simulink library "lib_AC_MGES"  (R2026a)
settings: Solver=VariableStepAuto
undefined symbols (not defined in the file): block_buses, block_fref, block_idx, block_toM, buses_lf, c_fd, c_kd1, c_kq1, c_kq2, fref, gen_static_params, Lbiginv, Lppd_pu, Lppq_pu, op_MGES, Ps_lf, Sb, T_meas_safe
(part 1 of 2)
settings Model: Creator=atomas  LastModifiedBy=atomas

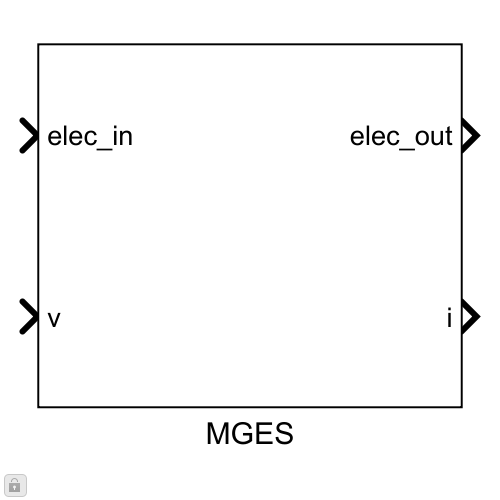
[thumbnail: Simulink's stored preview of the top-level diagram]
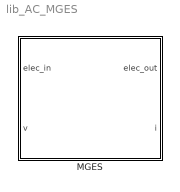
== system lib_AC_MGES ==
  MGES : Subsystem  mask(Synchronous machine){SGs_nodes=1, FBASE=50, D=0, H=3, Psimag_pu=0.8, Lssd_pu=0.1, Lssq_pu=0.1, Rs_pu=0.001, Lmd_pu=0.1, Lmq_pu=0.1, Rfd_pu=0.01, Lfd_pu=0.1, Rkd1_pu=1e6, Lkd1_pu=1e6, Rkd2_pu=1e6, Lkd2_pu=1e6, Rkq1_pu=1e6, Lkq1_pu=1e6, Rkq2_pu=1e6, Lkq2_pu=1e6, Rkq3_pu=1e6, Lkq3_pu=1e6, T_e=1, T_v=1, T_1=1, T_2=1, K_A=1, K_C=0, K_P=0, K_PR=1, K_IR=1, K_PM=1, K_IM=1, R_p=0.05, T_1g=1, T_2g=1, T_3=1, T_4=1, T_5=1, T_6=1, K_1=0, K_3=0, K_5=0, T_w1=1, T_w2=1, T_9=1, M=1, K_S1=0, T_1p=1, T_2p=1, T_3p=1, T_4p=1, T_7p=1, K_S2=1, K_S3=1, dynamic_stator=order 8, T_meas=0.01, cosn=1, T_w3=2}
      mask prompts: FBASE "Base frequency (Hz)"; D "Damping (pu)"; H "Inertia (s)"; Psimag_pu "Permanent flux (pu)"; Lssd_pu "Stator inductances (pu) Ld"; Lssq_pu "Stator inductances (pu) Lq"; Rs_pu "Stator resistances (pu)"; Lmd_pu "d-axis mutual inductance (pu)"; Lmq_pu "q-axis mutual inductance (pu)"; Rfd_pu "Excitation resistance (pu)"; Lfd_pu "Excitation inductance (pu)"; Rkd1_pu "d-axis damper resistance 1 (pu)"; Lkd1_pu "d-axis damper inductance 1 (pu)"; Rkd2_pu "d-axis damper resistance 2 (pu)"; Lkd2_pu "d-axis damper inductance 2 (pu)"; Rkq1_pu "q-axis damper resistance 1 (pu)"; Lkq1_pu "q-axis damper inductance 1 (pu)"; Rkq2_pu "q-axis damper resistance 2 (pu)"; Lkq2_pu "q-axis damper inductance 2 (pu)"; Rkq3_pu "q-axis damper resistance 3 (pu)"; Lkq3_pu "q-axis damper inductance 3 (pu)"; T_1p "T_1"; dynamic_stator "Electromagnetic complexity:"; T_meas "Governor speed measurement filter T_meas (s):"; cosn "Governor rated power factor cosn:"; T_w3 "PSS power washout time constant T_w3 (s):"
      mask help: Synchronous machine modelled in d-q reference frame.
      mask init:
      | [block_buses, block_idx, block_toM, block_fref, Lbiginv, Lssd_pu, Lssq_pu, Lmd_pu, Lmq_pu, Lfd_pu, Lkd1_pu, Lkd2_pu, Lkq1_pu, Lkq2_pu, Lkq3_pu, K_C, K_P, T_1, T_2, c_fd, c_kd1, Lppd_pu, c_kq1, c_kq2, Lppq_pu, stator_mode, use_Tmeas, use_PSS, use_LeadLag, use_KP, T_meas_safe, T_w3_safe, T_1_safe] = mask_init_MGES(gcb, Lssd_pu, Lssq_pu, Lmd_pu, Lmq_pu, Lfd_pu, Lkd1_pu, Lkd2_pu, Lkq1_pu, Lkq2_pu, Lkq3_pu, K_C, K_P, T_1, T_2, dynamic_stator, T_meas, K_S1, T_w3);
      mask Help: web([extractBefore(get_param(bdroot, 'filename'),gcs) 'Documentation/SM.html'])
      mask TypeOptions dynamic_stator: order 8 | order 4 | order 2
      mask DialogControl Params Prompt: Parameters
      mask DialogControl AVR Prompt: AVR
      mask DialogControl Gov Prompt: Speed governor
      mask DialogControl PSS Prompt: Power system stabiliser

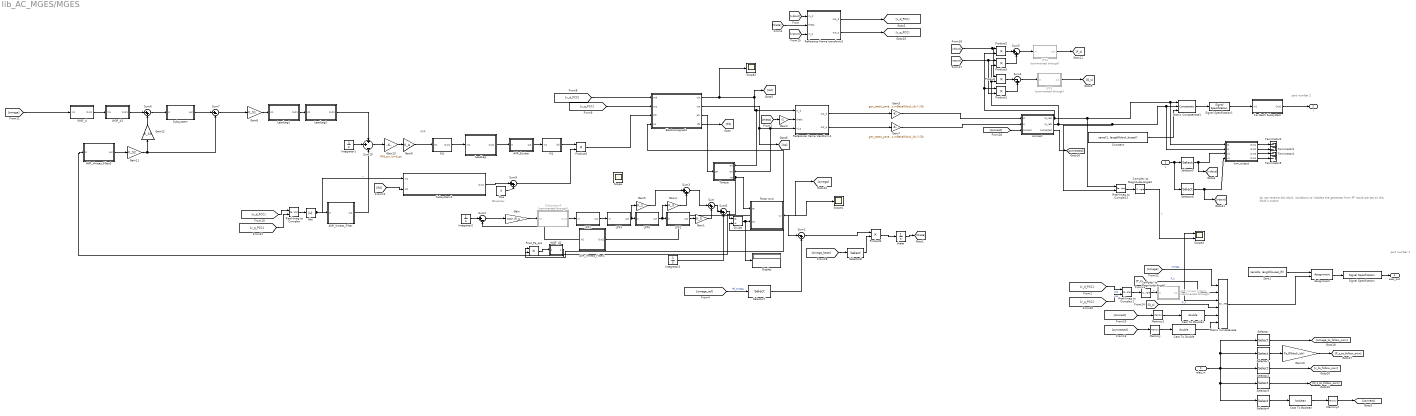
== system lib_AC_MGES/MGES ==
  note: Governor
  note: do not rename this block, conditions to initialise the generator from PF result are set on this block's output
  note: port number 1
  note: port number 2
  note: AVR
  elec_in : Inport
  v : Inport  Port=2
  AVR_Exciter : Subsystem  mask{T_s=T_e}
      mask prompts: T_s "Filter time constant"
  AVR_Vmeas_Filter : Subsystem  mask{T_r=T_v}
      mask prompts: T_r "Filter time constant"
  AVR_Vmeas_Filter1 : Subsystem  Variant=on
  AVR_Vmeas_Filter2 : Subsystem  Commented=through  mask{T_r=0.01}
      mask prompts: T_r "Filter time constant"
      mask Display:
      | try
      |     dpoly(1, [T_r, 1])
      | catch
      | end
  AVR_Vmeas_Filter3 : Subsystem  mask{T_r=T_7p}
      mask prompts: T_r "Filter time constant"
  Abs : Abs  SaturateOnIntegerOverflow=off
  Assignment : Assignment  NumberOfDimensions=2  DiagnosticForDimensions=Warning  IndexOptions=Assign all,Index vector (dialog)  Indices=1,block_idx  OutputSizes=1,1
  Cast To Boolean : DataTypeConversion  OutDataTypeStr=boolean  SaturateOnIntegerOverflow=off  RndMeth=Floor
  Cast To Double : DataTypeConversion  OutDataTypeStr=double  SaturateOnIntegerOverflow=off  RndMeth=Floor
  Cast To Double1 : DataTypeConversion  OutDataTypeStr=double  SaturateOnIntegerOverflow=off  RndMeth=Floor
  Complex to Magnitude-Angle1 : ComplexToMagnitudeAngle  Output=Magnitude
  Complex to Magnitude-Angle2 : ComplexToMagnitudeAngle  Output=Magnitude
  Constant : Constant  Value=zeros(1, length(block_buses))  VectorParams1D=off
  Display : Display
  Divide : Product  Inputs=*/
  Electromagnetic : Subsystem  Variant=on
  For Each Subsystem : Subsystem  TreatAsAtomicUnit=on
  Gain : Gain  Gain=cosn./R_p
  Gain1 : Gain  Gain=K_5
  Gain10 : Gain  Gain=Ps_lf(block_idx)
  Gain11 : Gain  Gain=K_S2
  Gain12 : Gain  Gain=K_S3
  Gain13 : Gain  Gain=Rfd_pu./Lmd_pu
  Gain2 : Gain  Gain=-1
  Gain3 : Gain  Gain=gen_static_params.mBase(block_idx)'./Sb
  Gain4 : Gain  Gain=K_3
  Gain5 : Gain  Gain=K_1
  Gain6 : Gain  Gain=K_A
  Gain7 : Gain  Gain=gen_static_params.mBase(block_idx)'./Sb
  Gain8 : Gain  Gain=K_S1
  Integrator1 : Integrator  InitialCondition=op_MGES.Integrator1
  Integrator2 : Integrator  InitialCondition=op_MGES.Integrator2
  Integrator3 : Integrator  InitialCondition=op_MGES.Integrator3
  LPF1 : Subsystem  mask{T_s=T_6}
      mask prompts: T_s "Filter time constant"
  LPF2 : Subsystem  mask{T_s=T_3}
      mask prompts: T_s "Filter time constant"
  LPF3 : Subsystem  mask{T_s=T_4}
      mask prompts: T_s "Filter time constant"
  LPF4 : Subsystem  Commented=through  mask{T_s=0.01}
      mask prompts: T_s "Filter time constant"
      mask Display:
      | try
      |     dpoly(1, [T_s, 1])
      | catch
      | end
  LPF5 : Subsystem  Commented=through  mask{T_s=0.01}
      mask prompts: T_s "Filter time constant"
      mask Display:
      | try
      |     dpoly(1, [T_s, 1])
      | catch
      | end
  LPF6 : Subsystem  mask{T_s=T_5}
      mask prompts: T_s "Filter time constant"
  LeadLag : Subsystem  Variant=on
  LeadLag1 : Subsystem  mask{T_2=T_1p, T_1=T_2p}
      mask help:
      | Transfer function:
      |
      |   1 + sT_2
      | ---------------
      |   1 + sT_1
  LeadLag2 : Subsystem  mask{T_2=T_3p, T_1=T_4p}
      mask help:
      | Transfer function:
      |
      |   1 + sT_2
      | ---------------
      |   1 + sT_1
  Matrix Concatenate : Concatenate  NumInputs=6  Mode=Multidimensional array
  Matrix Concatenate1 : Concatenate  NumInputs=3  Mode=Multidimensional array
  Memory : Memory  InitialCondition=1
  Memory1 : Memory  InitialCondition=1
  Memory2 : Memory  InitialCondition=1
  One : Constant  Value=0  OutDataTypeStr=Inherit: Inherit via back propagation
  PI1 : Subsystem
  PI2 : Subsystem
  Prod_Pe_pss : Product
  Product{,1..5} (6 alike) : Product
  Real-Imag to Complex : RealImagToComplex
  Real-Imag to Complex1 : RealImagToComplex
  Real-Imag to Complex2 : RealImagToComplex
  Reference frame transform1 : Subsystem
  Reference frame transform3 : Subsystem
  Rotor axis : Subsystem
  Scope : Scope
      settings: ActiveDisplayYMinimum=-1  ActiveDisplayYMaximum=1  DataLoggingVariableName=ScopeData13
  Scope1 : Scope
      settings: ActiveDisplayYMinimum=-0.058141408811601208  ActiveDisplayYMaximum=2.1702525958532117  DataLoggingVariableName=ScopeData3
  Scope2 : Scope
      settings: ActiveDisplayYMinimum=-0.402690614368146  ActiveDisplayYMaximum=1.3038964261892889  DataLoggingVariableName=ScopeData9
  Scope3 : Scope  NumInputPorts=2
      settings: ActiveDisplayYMinimum=0.29123  ActiveDisplayYMaximum=1.9416  DataLoggingVariableName=ScopeData3
  Selector : Selector  NumberOfDimensions=2  InputPortWidth=3  IndexOptions=Index vector (dialog),Index vector (dialog)  Indices=1,block_idx  OutputSizes=1,1
  Selector1 : Selector  NumberOfDimensions=2  InputPortWidth=3  IndexOptions=Index vector (dialog),Index vector (dialog)  Indices=2,block_idx  OutputSizes=1,1
  Selector2 : Selector  NumberOfDimensions=2  InputPortWidth=3  IndexOptions=Index vector (dialog),Index vector (dialog)  Indices=3,block_idx  OutputSizes=1,1
  Selector3 : Selector  NumberOfDimensions=2  InputPortWidth=3  IndexOptions=Index vector (dialog),Index vector (dialog)  Indices=4,block_idx  OutputSizes=1,1
  Selector4 : Selector  NumberOfDimensions=2  InputPortWidth=3  IndexOptions=Index vector (dialog),Index vector (dialog)  Indices=5,block_idx  OutputSizes=1,1
  Selector5 : Selector  NumberOfDimensions=2  InputPortWidth=3  IndexOptions=Index vector (dialog),Index vector (dialog)  Indices=1,block_buses  OutputSizes=1,1
  Selector6 : Selector  NumberOfDimensions=2  InputPortWidth=3  IndexOptions=Index vector (dialog),Index vector (dialog)  Indices=2,block_buses  OutputSizes=1,1
  Selector7 : Selector  InputPortWidth=length(fref.ref_units)  IndexOptions=Index vector (dialog)  Indices=block_fref  OutputSizes=1
  Selector8 : Selector  InputPortWidth=length(fref.ref_units)  IndexOptions=Index vector (dialog)  Indices=block_fref  OutputSizes=1
  Signal Specification : SignalSpecification  Dimensions=[6 length(buses_lf)]
  Signal Specification1 : SignalSpecification  Dimensions=[3 length(block_buses)]
  Subsystem : Subsystem
  Subsystem1 : Subsystem  Variant=on
  Subsystem4 : Subsystem  Commented=through  mask{T_2=T_2, T_1=T_1}
      mask help:
      | Transfer function:
      |
      |   1 + sT_2
      | ---------------
      |   1 + sT_1
  Sum{,3,5..6,8..9} (6 alike) : Sum  Inputs=|++
  Sum1 : Sum  Inputs=|-+
  Sum10 : Sum  Inputs=+|+|-
  Sum2 : Sum  Inputs=|+-
  Sum4 : Sum  Inputs=|-+
  Sum7 : Sum  Inputs=|+-
  Terminator{2..5} (4 alike) : Terminator
  Torque : Subsystem
      settings: PortSchema="{\"entries\":[{\"content\":{\"sides\":[{\"content\":{\"connectorIds\":[\"In1\"]},\"type\":\"ConnectorPlacement.EquallySpacedRectSide\",\"uuid\":\"b7abd3bc-22dd-4669-aa40-98bc76884565\"},{\"content\":{\"connectorIds\":[\"In2\",\"In3\",\"Out1\"],\"side\":\"RIGHT\"},\"type\":\"ConnectorPlacement.EquallySpacedRectSide\",\"uuid\":\"e9abb552-b46d-48ed-aa1f-0e9dac604fea\"},{\"content\":{\"connectorIds\":[],\"side\":\"TOP\"},\"type\":\"ConnectorPlacement.EquallySpacedRectSide\",\"uuid\":\"4b14997d-8f32-4cfb-8a1b-18cffb093d28\"}]},\"type\":\"ConnectorPlacement.EquallySpacedConnector\",\"uuid\":\"d6624493-e930-4f0d-8cbe-17f96cb72edc\"}],\"packageUris\":[\"http://schema.mathworks.com/mf0/Connector/R2020b\"],\"version\":\"1.0\"}"
  WOF_d : Subsystem
  WOF_d1 : Subsystem
  WOF_d2 : Subsystem  Variant=on
  Zero1 : Constant  Value=zeros(6, length(buses_lf))  VectorParams1D=off  OutDataTypeStr=Inherit: Inherit via back propagation
  connect : Subsystem
  theta : Integrator  InitialCondition=op_MGES.theta  UpperSaturationLimit=2*pi  LowerSaturationLimit=0
  trim_output : Subsystem
  elec_out : Outport
  i : Outport  Port=2
  wires:
  Subsystem1/1(Out1) -> Sum9/1
  [ifd] -> Subsystem1/2(In2)
  AVR_Vmeas_Filter/1(out) -> Sum10/3
  LeadLag/1(Out1) -> AVR_Exciter/1(in)
  PI2/1(Out1) -> LeadLag/1(In1)
  WOF_d2/1(Out1) -> AVR_Vmeas_Filter3/1(in)
  AVR_Vmeas_Filter1/1(Out1) -> Sum2/2
  Rotor axis/1(wr) -> AVR_Vmeas_Filter1/1(In1), Electromagnetic/4(ws), [omega], Scope1/1, Sum1/1, Divide/2, Prod_Pe_pss/2
  LPF5/1(out) -> [Q_s]
  Reference frame transform1/2(out_q) -> Gain7/1
  Product/1 -> Sum4/1
  Product1/1 -> Sum4/2
  theta/1 -> [theta]
  Gain2/1 -> Reference frame transform1/2(theta)
  [theta] -> Reference frame transform3/2(theta)
  LPF6/1(out) -> Gain4/1, LPF1/1(in)
  [theta] -> Gain2/1
  LPF2/1(out) -> LPF3/1(in)
  Sum4/1 -> LPF5/1(in)
  Sum5/1 -> LPF4/1(in)
  Product3/1 -> Sum5/2
  [omega_ref] -> Selector7/1  "ref_omega"
  Product2/1 -> Sum5/1
  Reference frame transform1/1(out_d) -> Gain3/1
  Subsystem4/1(Out1) -> LPF2/1(in)
  LPF4/1(out) -> [P_s]
  [P_s] -> Matrix Concatenate/2  "P_s"
  [omega] -> Matrix Concatenate/1  "omega"
  Complex to Magnitude-Angle1/1 -> AVR_Vmeas_Filter2/1(in)  "v"
  [Q_s] -> Matrix Concatenate/4  "Q_s"
  Selector3/1 -> [Q_s_to_follow_own]
  Selector/1 -> [omega_to_follow_own]
  Selector1/1 -> Gain10/1
  Selector2/1 -> [v_to_follow_own]
  [connect] -> Memory1/1
  [connected] -> Memory/1
  Cast To Double1/1 -> Matrix Concatenate/5
  Cast To Double/1 -> Matrix Concatenate/6
  Real-Imag to Complex1/1 -> Complex to Magnitude-Angle1/1
  [vdout] -> Product/1, Product2/1
  [vqout] -> Product3/1, Product1/2
  [v_d_PCC] -> Real-Imag to Complex1/1  "vod"
  [v_q_PCC] -> Real-Imag to Complex1/2  "voq"
  connect/3(connected) -> [connected]
  [connect] -> connect/3(connect)
  connect/1(id_real) -> Real-Imag to Complex2/1, trim_output/1(id), Matrix Concatenate1/1, Product1/1, Product2/2
  Selector4/1 -> Cast To Boolean/1
  Cast To Boolean/1 -> Memory2/1
  Zero1/1 -> Assignment/1
  Signal Specification/1 -> elec_out/1
  elec_in/1 -> Selector4/1, Selector3/1, Selector2/1, Selector1/1, Selector/1
  Assignment/1 -> Signal Specification/1
  Matrix Concatenate/1 -> Assignment/2
  Matrix Concatenate1/1 -> Signal Specification1/1
  Signal Specification1/1 -> For Each Subsystem/1(In1)
  Constant/1 -> Matrix Concatenate1/3
  For Each Subsystem/1(Out1) -> i/1
  connect/2(iq_real) -> Product3/2, Product/2, Real-Imag to Complex2/2, trim_output/2(iq), Matrix Concatenate1/2
  trim_output/3(Out3) -> Terminator4/1
  trim_output/1(Out1) -> Terminator2/1
  trim_output/4(Out4) -> Terminator5/1
  trim_output/2(Out2) -> Terminator3/1
  v/1 -> Selector6/1, Selector5/1
  Selector5/1 -> [vdout], trim_output/3(vd)
  Selector6/1 -> [vqout], trim_output/4(vq)
  [vqout] -> Reference frame transform3/3(in_q)
  [vdout] -> Reference frame transform3/1(in_d)
  Reference frame transform3/1(out_d) -> [v_d_PCC]
  Reference frame transform3/2(out_q) -> [v_q_PCC]
  Memory/1 -> Cast To Double/1
  Gain10/1 -> [P_s_to_follow_own]
  Memory1/1 -> Cast To Double1/1
  Memory2/1 -> [connect]
  Selector7/1 -> Sum1/2
  Selector8/1 -> Product4/2
  [omega_base] -> Selector8/1
  Product4/1 -> theta/1
  Sum1/1 -> Product4/1
  Gain/1 -> Subsystem4/1(In1)
  Sum2/1 -> Gain/1
  Integrator1/1 -> Sum10/2
  Gain6/1 -> PI2/1(In1)
  [v_d_PCC] -> Real-Imag to Complex/1
  Abs/1 -> AVR_Vmeas_Filter/1(in), Subsystem1/1(In1)  "v"
  [v_q_PCC] -> Real-Imag to Complex/2
  Real-Imag to Complex/1 -> Abs/1
  AVR_Vmeas_Filter2/1(out) -> Matrix Concatenate/3, Scope3/1
  Real-Imag to Complex2/1 -> Complex to Magnitude-Angle2/1
  Complex to Magnitude-Angle2/1 -> Scope3/2  "v"
  Electromagnetic/2(isq) -> [isq], Torque/3(isq), Reference frame transform1/3(in_q)
  Electromagnetic/1(isd) -> Scope2/1, Reference frame transform1/1(in_d), Torque/2(isd), [isd]
  [v_d_PCC] -> Electromagnetic/1(vsd)
  [v_q_PCC] -> Electromagnetic/2(vsq)
  Electromagnetic/3(psi) -> Torque/1(psi)
  Electromagnetic/4(ifd) -> [ifd]
  AVR_Exciter/1(out) -> PI1/1(In1)
  PI1/1(vfd) -> Product5/1
  LPF3/1(out) -> Gain5/1, LPF6/1(in)
  LPF1/1(out) -> Gain1/1
  Gain1/1 -> Sum/2
  Sum3/1 -> Sum/1
  Gain4/1 -> Sum3/2
  Gain5/1 -> Sum3/1
  Gain3/1 -> connect/1(id)
  Gain7/1 -> connect/2(iq)
  WOF_d/1(Out1) -> WOF_d1/1(In1)
  Gain8/1 -> LeadLag1/1(In1)
  LeadLag1/1(Out1) -> LeadLag2/1(In1)
  [omega] -> WOF_d/1(In1)
  WOF_d1/1(Out1) -> Sum6/1
  Sum6/1 -> Subsystem/1(in)
  Subsystem/1(out) -> Sum7/1
  Sum7/1 -> Gain8/1
  Gain12/1 -> Sum6/2
  Gain11/1 -> Sum7/2, Gain12/1
  AVR_Vmeas_Filter3/1(out) -> Gain11/1
  Integrator2/1 -> Sum2/1
  Torque/1(te) -> Rotor axis/1(te), Prod_Pe_pss/1
  Sum10/1 -> Gain13/1
  Gain13/1 -> Gain6/1
  Sum/1 -> Sum8/1
  Sum8/1 -> Divide/1
  Integrator3/1 -> Sum8/2
  LeadLag2/1(Out1) -> Sum10/1
  Divide/1 -> Display/1, Rotor axis/2(tm)
  Product5/1 -> Electromagnetic/3(vfd)
  Sum9/1 -> Product5/2
  One/1 -> Sum9/2
  Prod_Pe_pss/1 -> WOF_d2/1(In1)

== system lib_AC_MGES/MGES/AVR_Exciter ==
  in : Inport
  Gain : Gain  Gain=1./T_s
  Sum4 : Sum  Inputs=|+-
  x_a : Integrator  InitialCondition=op_MGES.AVR_Exciter_x_a
  out : Outport
  wires:
  Gain/1 -> x_a/1
  Sum4/1 -> Gain/1
  in/1 -> Sum4/1
  x_a/1 -> out/1, Sum4/2

== system lib_AC_MGES/MGES/AVR_Vmeas_Filter ==
  in : Inport
  Gain : Gain  Gain=1./T_r
  Sum4 : Sum  Inputs=|+-
  x_a : Integrator  InitialCondition=op_MGES.AVR_Vmeas_Filter_x_a
  out : Outport
  wires:
  Gain/1 -> x_a/1
  Sum4/1 -> Gain/1
  in/1 -> Sum4/1
  x_a/1 -> out/1, Sum4/2

== system lib_AC_MGES/MGES/AVR_Vmeas_Filter1 ==
  note: 1) Add Subsystem or Model blocks as valid variant choices.
      | 2) You cannot connect blocks at this level. At simulation, connectivity is automatically
      | determined, based on the active variant and port name matching.
  In1 : Inport
  Active : Subsystem  VariantControl=use_Tmeas == 1
  Bypass : Subsystem  VariantControl=(default)
  Out1 : Outport

== system lib_AC_MGES/MGES/AVR_Vmeas_Filter2 ==
  in : Inport
  Gain : Gain  Gain=1./T_r
  Sum4 : Sum  Inputs=|+-
  x_a : Integrator  InitialCondition=op_MGES.AVR_Vmeas_Filter2_x_a
  out : Outport
  wires:
  Gain/1 -> x_a/1
  Sum4/1 -> Gain/1
  in/1 -> Sum4/1
  x_a/1 -> out/1, Sum4/2

== system lib_AC_MGES/MGES/AVR_Vmeas_Filter3 ==
  in : Inport
  Gain : Gain  Gain=1./T_r
  Sum4 : Sum  Inputs=|+-
  x_a : Integrator  InitialCondition=op_MGES.AVR_Vmeas_Filter3_x_a
  out : Outport
  wires:
  x_a/1 -> Sum4/2, out/1
  in/1 -> Sum4/1
  Sum4/1 -> Gain/1
  Gain/1 -> x_a/1

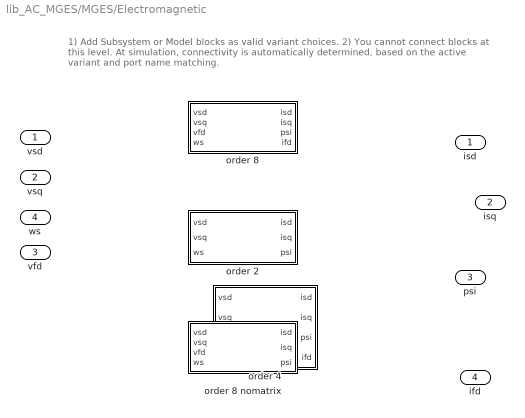
== system lib_AC_MGES/MGES/Electromagnetic ==
  note: 1) Add Subsystem or Model blocks as valid variant choices.
      | 2) You cannot connect blocks at this level. At simulation, connectivity is automatically
      | determined, based on the active variant and port name matching.
  vsd : Inport
  vsq : Inport  Port=2
  vfd : Inport  Port=3
  ws : Inport  Port=4
  order 2 : Subsystem  VariantControl=stator_mode == 2
  order 4 : Subsystem  VariantControl=stator_mode == 4
  order 8 : Subsystem  VariantControl=(default)
  order 8 nomatrix : Subsystem  VariantControl=stator_mode == 1  mask{Lssd_pu=Lssd_pu, Lssq_pu=Lssq_pu, Lmd_pu=Lmd_pu, Lmq_pu=Lmq_pu, Lfd_pu=Lfd_pu, Lkd1_pu=Lkd1_pu, Lkd2_pu=Lkd2_pu, Lkq1_pu=Lkq1_pu, Lkq2_pu=Lkq2_pu, Lkq3_pu=Lkq3_pu}
      mask init:
      | Matrix_flux_to_i = mask_init_order8_nomatrix(Lssd_pu, Lssq_pu, Lmd_pu, Lmq_pu, Lfd_pu, Lkd1_pu, Lkd2_pu, Lkq1_pu, Lkq2_pu, Lkq3_pu);
  isd : Outport
  isq : Outport  Port=2
  psi : Outport  Port=3
  ifd : Outport  Port=4

== system lib_AC_MGES/MGES/For Each Subsystem ==
  In1 : Inport  Partition=on  PartitionDimension=1  PartitionWidth=1  PartitionOffset=0
  For Each : ForEach  DisableCoverage=on
  State-Space : StateSpace  A=[]  B=[]  C=[]  D=block_toM  InitialCondition=0  ParameterTunability=Optimized
  Transpose : Math  Operator=transpose
  Transpose1 : Math  Operator=transpose
  Out1 : Outport  ConcatenationDimension=1
  wires:
  Transpose1/1 -> Out1/1
  In1/1 -> Transpose/1
  Transpose/1 -> State-Space/1
  State-Space/1 -> Transpose1/1

== system lib_AC_MGES/MGES/LPF1 ==
  in : Inport
  Gain : Gain  Gain=1./T_s
  Sum4 : Sum  Inputs=|+-
  x_a : Integrator  InitialConditionSource=external  InitialCondition=op_MGES.LPF1_x_a
  out : Outport
  wires:
  Gain/1 -> x_a/1
  Sum4/1 -> Gain/1
  in/1 -> x_a/2, Sum4/1
  x_a/1 -> out/1, Sum4/2

== system lib_AC_MGES/MGES/LPF2 ==
  in : Inport
  Gain : Gain  Gain=1./T_s
  Sum4 : Sum  Inputs=|+-
  x_a : Integrator  InitialConditionSource=external  InitialCondition=op_MGES.LPF2_x_a
  out : Outport
  wires:
  Gain/1 -> x_a/1
  Sum4/1 -> Gain/1
  in/1 -> x_a/2, Sum4/1
  x_a/1 -> out/1, Sum4/2

== system lib_AC_MGES/MGES/LPF3 ==
  in : Inport
  Gain : Gain  Gain=1./T_s
  Sum4 : Sum  Inputs=|+-
  x_a : Integrator  InitialConditionSource=external  InitialCondition=op_MGES.LPF3_x_a
  out : Outport
  wires:
  Gain/1 -> x_a/1
  Sum4/1 -> Gain/1
  in/1 -> x_a/2, Sum4/1
  x_a/1 -> out/1, Sum4/2

== system lib_AC_MGES/MGES/LPF4 ==
  in : Inport
  Gain : Gain  Gain=1./T_s
  Sum4 : Sum  Inputs=|+-
  x_a : Integrator  InitialCondition=op_MGES.LPF4_x_a
  out : Outport
  wires:
  x_a/1 -> Sum4/2, out/1
  in/1 -> Sum4/1
  Sum4/1 -> Gain/1
  Gain/1 -> x_a/1

== system lib_AC_MGES/MGES/LPF5 ==
  in : Inport
  Gain : Gain  Gain=1./T_s
  Sum4 : Sum  Inputs=|+-
  x_a : Integrator  InitialCondition=op_MGES.LPF5_x_a
  out : Outport
  wires:
  Gain/1 -> x_a/1
  Sum4/1 -> Gain/1
  in/1 -> Sum4/1
  x_a/1 -> out/1, Sum4/2

== system lib_AC_MGES/MGES/LPF6 ==
  in : Inport
  Gain : Gain  Gain=1./T_s
  Sum4 : Sum  Inputs=|+-
  x_a : Integrator  InitialConditionSource=external  InitialCondition=op_MGES.LPF6_x_a
  out : Outport
  wires:
  Gain/1 -> x_a/1
  Sum4/1 -> Gain/1
  in/1 -> x_a/2, Sum4/1
  x_a/1 -> out/1, Sum4/2

== system lib_AC_MGES/MGES/LeadLag ==
  note: 1) Add Subsystem or Model blocks as valid variant choices.
      | 2) You cannot connect blocks at this level. At simulation, connectivity is automatically
      | determined, based on the active variant and port name matching.
  In1 : Inport
  Active : Subsystem  VariantControl=use_LeadLag == 1
  Bypass : Subsystem  VariantControl=(default)
  Out1 : Outport

== system lib_AC_MGES/MGES/LeadLag1 ==
  In1 : Inport
  Gain : Gain  Gain=1./T_1
  Gain2 : Gain  Gain=T_2./T_1
  Sum : Sum  Inputs=|+-
  Sum1 : Sum  Inputs=++|
  x_f : Integrator  InitialConditionSource=external  InitialCondition=op_MGES.LeadLag1_x_f
  Out1 : Outport
  wires:
  x_f/1 -> Sum1/2, Sum/2
  Gain/1 -> x_f/1
  Sum/1 -> Gain/1, Gain2/1
  Gain2/1 -> Sum1/1
  Sum1/1 -> Out1/1
  In1/1 -> x_f/2, Sum/1

== system lib_AC_MGES/MGES/LeadLag2 ==
  In1 : Inport
  Gain : Gain  Gain=1./T_1
  Gain2 : Gain  Gain=T_2./T_1
  Sum : Sum  Inputs=|+-
  Sum1 : Sum  Inputs=++|
  x_f : Integrator  InitialConditionSource=external  InitialCondition=op_MGES.LeadLag2_x_f
  Out1 : Outport
  wires:
  In1/1 -> Sum/1, x_f/2
  Sum1/1 -> Out1/1
  Gain2/1 -> Sum1/1
  Sum/1 -> Gain2/1, Gain/1
  Gain/1 -> x_f/1
  x_f/1 -> Sum/2, Sum1/2

== system lib_AC_MGES/MGES/PI1 ==
  In1 : Inport
  Gain1 : Gain  Gain=K_IM ~= 0
  Gain4 : Gain  Gain=K_PM
  Gain5 : Gain  Gain=K_IM
  Integrator : Integrator  InitialCondition=op_MGES.PI1_Integrator
  Sum7 : Sum  Inputs=|++
  vfd : Outport
  wires:
  Integrator/1 -> Gain1/1
  Gain4/1 -> Sum7/1
  Sum7/1 -> vfd/1
  In1/1 -> Gain4/1, Gain5/1
  Gain5/1 -> Integrator/1
  Gain1/1 -> Sum7/2

== system lib_AC_MGES/MGES/PI2 ==
  In1 : Inport
  Gain1 : Gain  Gain=K_IR ~= 0
  Gain4 : Gain  Gain=K_PR
  Gain5 : Gain  Gain=K_IR
  Integrator : Integrator  InitialCondition=op_MGES.PI2_Integrator
  Sum7 : Sum  Inputs=|++
  Out1 : Outport
  wires:
  Integrator/1 -> Gain1/1
  Gain4/1 -> Sum7/1
  Sum7/1 -> Out1/1
  In1/1 -> Gain4/1, Gain5/1
  Gain5/1 -> Integrator/1
  Gain1/1 -> Sum7/2

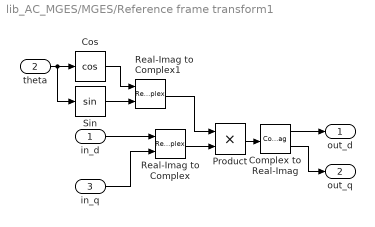
== system lib_AC_MGES/MGES/Reference frame transform1 ==
  in_d : Inport
  theta : Inport  Port=2
  in_q : Inport  Port=3
  Complex to Real-Imag : ComplexToRealImag
  Cos : Trigonometry  SCDEnableBlockLinearizationSpecification=on  Operator=cos
  Product : Product
  Real-Imag to Complex : RealImagToComplex
  Real-Imag to Complex1 : RealImagToComplex
  Sin : Trigonometry  SCDEnableBlockLinearizationSpecification=on
  out_d : Outport
  out_q : Outport  Port=2
  wires:
  in_d/1 -> Real-Imag to Complex/1
  in_q/1 -> Real-Imag to Complex/2
  Complex to Real-Imag/1 -> out_d/1
  Sin/1 -> Real-Imag to Complex1/2
  Cos/1 -> Real-Imag to Complex1/1
  theta/1 -> Cos/1, Sin/1
  Product/1 -> Complex to Real-Imag/1
  Real-Imag to Complex/1 -> Product/2
  Real-Imag to Complex1/1 -> Product/1
  Complex to Real-Imag/2 -> out_q/1

== system lib_AC_MGES/MGES/Reference frame transform3 ==
  in_d : Inport
  theta : Inport  Port=2
  in_q : Inport  Port=3
  Complex to Real-Imag : ComplexToRealImag
  Cos : Trigonometry  SCDEnableBlockLinearizationSpecification=on  Operator=cos
  Product : Product
  Real-Imag to Complex : RealImagToComplex
  Real-Imag to Complex1 : RealImagToComplex
  Sin : Trigonometry  SCDEnableBlockLinearizationSpecification=on
  out_d : Outport
  out_q : Outport  Port=2
  wires:
  Complex to Real-Imag/2 -> out_q/1
  Real-Imag to Complex1/1 -> Product/1
  Real-Imag to Complex/1 -> Product/2
  Product/1 -> Complex to Real-Imag/1
  theta/1 -> Sin/1, Cos/1
  Cos/1 -> Real-Imag to Complex1/1
  Sin/1 -> Real-Imag to Complex1/2
  Complex to Real-Imag/1 -> out_d/1
  in_q/1 -> Real-Imag to Complex/2
  in_d/1 -> Real-Imag to Complex/1

== system lib_AC_MGES/MGES/Rotor axis ==
  te : Inport
  tm : Inport  Port=2
  Gain : Gain  Gain=1./(2*H)
  Gain1 : Gain  Gain=D
  Sum1 : Sum  Inputs=+|-|-  InputSameDT=on  SaturateOnIntegerOverflow=on  OutDataTypeStr=Inherit: Same as first input
  \omega_r : Integrator  InitialCondition=op_MGES.Rotor_axis_omega_r  UpperSaturationLimit=2*pi  LowerSaturationLimit=0
  wr : Outport  VectorParamsAs1DForOutWhenUnconnected=off
  wires:
  tm/1 -> Sum1/1
  \omega_r/1 -> wr/1, Gain1/1
  te/1 -> Sum1/2
  Sum1/1 -> Gain/1
  Gain/1 -> \omega_r/1
  Gain1/1 -> Sum1/3

== system lib_AC_MGES/MGES/Subsystem ==
  in : Inport
  LPF1 : Subsystem  mask{T_s=T_9}
      mask prompts: T_s "Filter time constant"
  LPF2 : Subsystem  mask{T_s=T_9}
      mask prompts: T_s "Filter time constant"
  LPF3 : Subsystem  mask{T_s=T_9}
      mask prompts: T_s "Filter time constant"
  LPF4 : Subsystem  mask{T_s=T_9}
      mask prompts: T_s "Filter time constant"
  LPF7 : Subsystem  mask{T_s=T_9}
      mask prompts: T_s "Filter time constant"
  out : Outport
  wires:
  LPF2/1(out) -> LPF3/1(in)
  LPF3/1(out) -> LPF4/1(in)
  LPF7/1(out) -> LPF1/1(in)
  LPF4/1(out) -> out/1
  LPF1/1(out) -> LPF2/1(in)
  in/1 -> LPF7/1(in)

== system lib_AC_MGES/MGES/Subsystem1 ==
  note: 1) Add Subsystem or Model blocks as valid variant choices.
      | 2) You cannot connect blocks at this level. At simulation, connectivity is automatically
      | determined, based on the active variant and port name matching.
  In1 : Inport
  In2 : Inport  Port=2
  Active : Subsystem  VariantControl=use_KP == 1
  Bypass : Subsystem  VariantControl=(default)
  Out1 : Outport

== system lib_AC_MGES/MGES/Subsystem4 ==
  In1 : Inport
  Gain : Gain  Gain=1./T_1
  Gain2 : Gain  Gain=T_2./T_1
  Sum : Sum  Inputs=|+-
  Sum1 : Sum  Inputs=++|
  x_f : Integrator  InitialCondition=op_MGES.Subsystem4_x_f
  Out1 : Outport
  wires:
  x_f/1 -> Sum1/2, Sum/2
  Gain/1 -> x_f/1
  Sum/1 -> Gain/1, Gain2/1
  Gain2/1 -> Sum1/1
  Sum1/1 -> Out1/1
  In1/1 -> Sum/1

== system lib_AC_MGES/MGES/Torque ==
  psi : Inport
  isd : Inport  Port=2
  isq : Inport  Port=3
  Product1 : Product
  Product2 : Product
  Selector : Selector  NumberOfDimensions=2  InputPortWidth=9  IndexOptions=Index vector (dialog),Select all  Indices=[1],1  OutputSizes=1,1
  Selector1 : Selector  NumberOfDimensions=2  InputPortWidth=9  IndexOptions=Index vector (dialog),Select all  Indices=[2],1  OutputSizes=1,1
  Sum : Sum  Inputs=+||-
  te : Outport  VectorParamsAs1DForOutWhenUnconnected=off
  wires:
  Product1/1 -> Sum/1
  Sum/1 -> te/1
  Selector/1 -> Product1/1  "psistatordq"
  psi/1 -> Selector1/1, Selector/1
  Product2/1 -> Sum/2
  isq/1 -> Product1/2
  isd/1 -> Product2/1
  Selector1/1 -> Product2/2  "psistatordq"

== system lib_AC_MGES/MGES/WOF_d ==
  In1 : Inport
  Gain : Gain  Gain=1./T_w1
  I : Integrator  InitialConditionSource=external  InitialCondition=op_MGES.WOF_d_I
  Sum : Sum  Inputs=+-|
  Sum4 : Sum  Inputs=|+-
  Out1 : Outport
  wires:
  Sum/1 -> Out1/1
  I/1 -> Sum/2, Sum4/2
  In1/1 -> Sum4/1, Sum/1, I/2
  Sum4/1 -> Gain/1
  Gain/1 -> I/1

== system lib_AC_MGES/MGES/WOF_d1 ==
  In1 : Inport
  Gain : Gain  Gain=1./T_w2
  I : Integrator  InitialConditionSource=external  InitialCondition=op_MGES.WOF_d1_I
  Sum : Sum  Inputs=+-|
  Sum4 : Sum  Inputs=|+-
  Out1 : Outport
  wires:
  Sum/1 -> Out1/1
  I/1 -> Sum/2, Sum4/2
  In1/1 -> Sum4/1, Sum/1, I/2
  Sum4/1 -> Gain/1
  Gain/1 -> I/1

== system lib_AC_MGES/MGES/WOF_d2 ==
  note: 1) Add Subsystem or Model blocks as valid variant choices.
      | 2) You cannot connect blocks at this level. At simulation, connectivity is automatically
      | determined, based on the active variant and port name matching.
  In1 : Inport
  Active : Subsystem  VariantControl=use_PSS == 1
  Bypass : Subsystem  VariantControl=(default)
  Out1 : Outport

== system lib_AC_MGES/MGES/connect ==
  id : Inport
  iq : Inport  Port=2
  connect : Inport  Port=3
  Switch : Switch  Criteria=u2 > Threshold  ZeroCross=off  SaturateOnIntegerOverflow=off  InputSameDT=off
  Switch1 : Switch  Criteria=u2 > Threshold  ZeroCross=off  SaturateOnIntegerOverflow=off  InputSameDT=off
  Zero1 : Constant  Value=0  VectorParams1D=off  OutDataTypeStr=Inherit: Inherit via back propagation
  Zero2 : Constant  Value=0  VectorParams1D=off  OutDataTypeStr=Inherit: Inherit via back propagation
  id_real : Outport
  iq_real : Outport  Port=2
  connected : Outport  Port=3  OutDataTypeStr=boolean
  wires:
  Switch/1 -> id_real/1
  Zero1/1 -> Switch/3
  id/1 -> Switch/1
  connect/1 -> connected/1, Switch1/2, Switch/2
  Switch1/1 -> iq_real/1
  iq/1 -> Switch1/1
  Zero2/1 -> Switch1/3

== system lib_AC_MGES/MGES/trim_output ==
  id : Inport
  iq : Inport  Port=2
  vd : Inport  Port=3
  vq : Inport  Port=4
  Out1 : Outport
  Out2 : Outport  Port=2
  Out3 : Outport  Port=3
  Out4 : Outport  Port=4
  wires:
  id/1 -> Out1/1
  vq/1 -> Out4/1
  vd/1 -> Out3/1
  iq/1 -> Out2/1

== system lib_AC_MGES/MGES/AVR_Vmeas_Filter1/Active ==
  In1 : Inport
  Impl : Subsystem  mask{T_r=T_meas_safe}
      mask prompts: T_r "Filter time constant"
  Out1 : Outport
  wires:
  Impl/1(out) -> Out1/1
  In1/1 -> Impl/1(in)

== system lib_AC_MGES/MGES/AVR_Vmeas_Filter1/Bypass ==
  In1 : Inport
  Out1 : Outport
  wires:
  In1/1 -> Out1/1

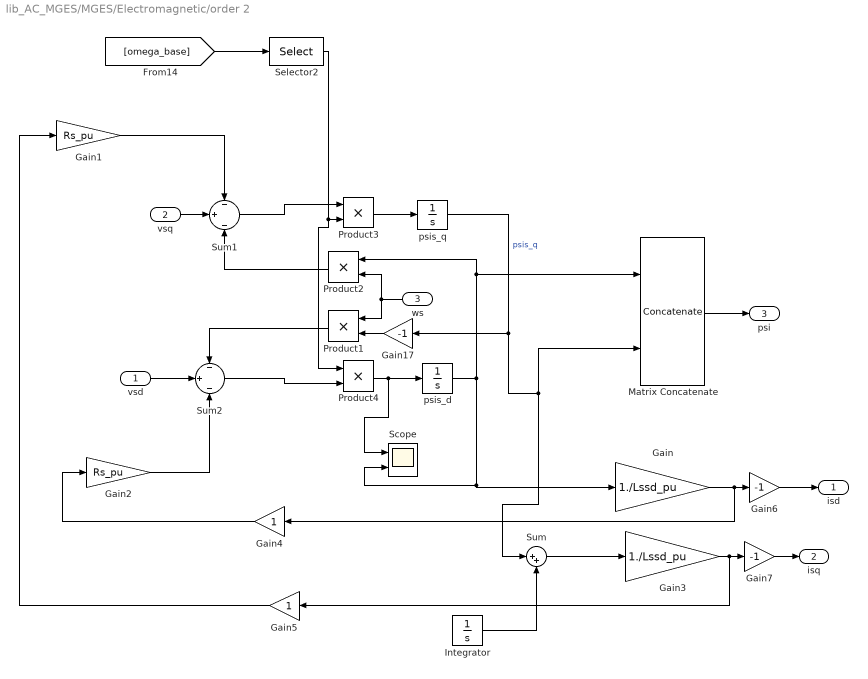
== system lib_AC_MGES/MGES/Electromagnetic/order 2 ==
  vsd : Inport
  vsq : Inport  Port=2
  ws : Inport  Port=3
  Gain : Gain  Gain=1./Lssd_pu
  Gain1 : Gain  Gain=Rs_pu
  Gain17 : Gain  Gain=-1
  Gain2 : Gain  Gain=Rs_pu
  Gain3 : Gain  Gain=1./Lssd_pu
  Gain4 : Gain
  Gain5 : Gain
  Gain6 : Gain  Gain=-1
  Gain7 : Gain  Gain=-1
  Integrator : Integrator  InitialCondition=op_MGES.Electromagnetic_order_2_Integrator
  Matrix Concatenate : Concatenate  Mode=Multidimensional array
  Product{1..4} (4 alike) : Product
  Scope : Scope  NumInputPorts=2
      settings: ActiveDisplayYMinimum=-176.647  ActiveDisplayYMaximum=19.6557
  Selector2 : Selector  InputPortWidth=length(fref.ref_units)  IndexOptions=Index vector (dialog)  Indices=block_fref  OutputSizes=1
  Sum : Sum  Inputs=|++
  Sum1 : Sum  Inputs=-|+|-  InputSameDT=on  SaturateOnIntegerOverflow=on  OutDataTypeStr=Inherit: Same as first input
  Sum2 : Sum  Inputs=-|+|-  InputSameDT=on  SaturateOnIntegerOverflow=on  OutDataTypeStr=Inherit: Same as first input
  psis_d : Integrator  InitialCondition=op_MGES.Electromagnetic_order_2_psis_d
  psis_q : Integrator  InitialCondition=op_MGES.Electromagnetic_order_2_psis_q
  isd : Outport  VectorParamsAs1DForOutWhenUnconnected=off
  isq : Outport  Port=2  VectorParamsAs1DForOutWhenUnconnected=off
  psi : Outport  Port=3  VectorParamsAs1DForOutWhenUnconnected=off
  wires:
  Product4/1 -> Scope/1, psis_d/1
  vsd/1 -> Sum2/2
  ws/1 -> Product1/1, Product2/2
  Matrix Concatenate/1 -> psi/1
  Product3/1 -> psis_q/1
  Sum1/1 -> Product3/1
  Product1/1 -> Sum2/1
  Product2/1 -> Sum1/3
  Sum2/1 -> Product4/2
  psis_q/1 -> Sum/1, Matrix Concatenate/2, Gain17/1  "psis_q"
  Gain1/1 -> Sum1/1
  [omega_base] -> Selector2/1
  vsq/1 -> Sum1/2
  Gain/1 -> Gain4/1, Gain6/1
  Gain2/1 -> Sum2/3
  Gain3/1 -> Gain5/1, Gain7/1
  Gain17/1 -> Product1/2
  Selector2/1 -> Product4/1, Product3/2
  Sum/1 -> Gain3/1
  Integrator/1 -> Sum/2
  Gain4/1 -> Gain2/1
  Gain5/1 -> Gain1/1
  psis_d/1 -> Product2/1, Matrix Concatenate/1, Gain/1, Scope/2
  Gain6/1 -> isd/1
  Gain7/1 -> isq/1

== system lib_AC_MGES/MGES/Electromagnetic/order 4 ==
  vsd : Inport
  vsq : Inport  Port=2
  vfd : Inport  Port=3
  ws : Inport  Port=4
  Stator circuit : Subsystem
  psi->i : Subsystem
  isd : Outport
  isq : Outport  Port=2
  psi : Outport  Port=3
  ifd : Outport  Port=4
  wires:
  psi->i/4(ifd) -> ifd/1
  psi->i/1(isd) -> isd/1
  vfd/1 -> Stator circuit/5(vfd)
  Stator circuit/1(psi) -> psi->i/1(psi), psi/1
  ws/1 -> Stator circuit/4(ws)
  vsq/1 -> Stator circuit/2(vsq)
  vsd/1 -> Stator circuit/1(vsd)
  psi->i/2(i) -> Stator circuit/3(i)
  psi->i/3(isq) -> isq/1

== system lib_AC_MGES/MGES/Electromagnetic/order 8 ==
  vsd : Inport
  vsq : Inport  Port=2
  vfd : Inport  Port=3
  ws : Inport  Port=4
  Stator circuit : Subsystem
  psi->i : Subsystem
  isd : Outport
  isq : Outport  Port=2
  psi : Outport  Port=3
  ifd : Outport  Port=4
  wires:
  psi->i/3(isq) -> isq/1
  psi->i/2(i) -> Stator circuit/3(i)
  vsd/1 -> Stator circuit/1(vsd)
  vsq/1 -> Stator circuit/2(vsq)
  ws/1 -> Stator circuit/4(ws)
  Stator circuit/1(psi) -> psi/1, psi->i/1(psi)
  vfd/1 -> Stator circuit/5(vfd)
  psi->i/1(isd) -> isd/1
  psi->i/4(ifd) -> ifd/1

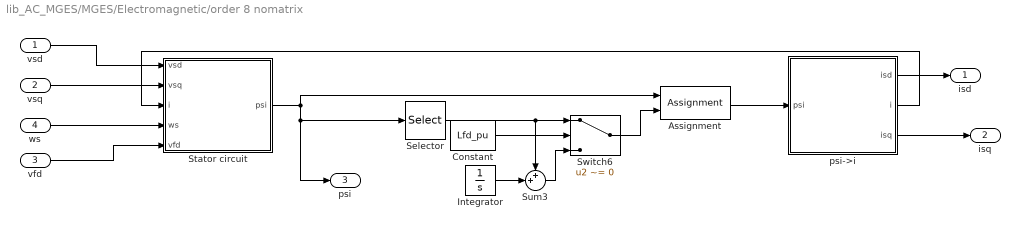
== system lib_AC_MGES/MGES/Electromagnetic/order 8 nomatrix ==
  vsd : Inport
  vsq : Inport  Port=2
  vfd : Inport  Port=3
  ws : Inport  Port=4
  Assignment : Assignment  NumberOfDimensions=2  DiagnosticForDimensions=Warning  IndexOptions=Index vector (dialog),Assign all  Indices=2,1  OutputSizes=1,1
  Constant : Constant  Value=Lfd_pu  VectorParams1D=off
  Integrator : Integrator  InitialCondition=op_MGES.Electromagnetic_order_8_nomatrix_Integrator
  Selector : Selector  NumberOfDimensions=2  InputPortWidth=3  IndexOptions=Index vector (dialog),Select all  Indices=2,1  OutputSizes=1,1
  Stator circuit : Subsystem
  Sum3 : Sum  Inputs=++|
  Switch6 : Switch  Criteria=u2 ~= 0  SaturateOnIntegerOverflow=off  InputSameDT=off
  psi->i : Subsystem
  isd : Outport
  isq : Outport  Port=2
  psi : Outport  Port=3
  wires:
  psi->i/3(isq) -> isq/1
  psi->i/2(i) -> Stator circuit/3(i)
  vsd/1 -> Stator circuit/1(vsd)
  vsq/1 -> Stator circuit/2(vsq)
  ws/1 -> Stator circuit/4(ws)
  Stator circuit/1(psi) -> psi/1, Selector/1, Assignment/1
  vfd/1 -> Stator circuit/5(vfd)
  psi->i/1(isd) -> isd/1
  Sum3/1 -> Switch6/3
  Constant/1 -> Switch6/2
  Integrator/1 -> Sum3/2
  Assignment/1 -> psi->i/1(psi)
  Selector/1 -> Sum3/1, Switch6/1
  Switch6/1 -> Assignment/2

== system lib_AC_MGES/MGES/LeadLag/Active ==
  In1 : Inport
  Impl : Subsystem
  Out1 : Outport
  wires:
  Impl/1(Out1) -> Out1/1
  In1/1 -> Impl/1(In1)

== system lib_AC_MGES/MGES/LeadLag/Bypass ==
  In1 : Inport
  Out1 : Outport
  wires:
  In1/1 -> Out1/1

== system lib_AC_MGES/MGES/Subsystem/LPF1 ==
  in : Inport
  Gain : Gain  Gain=1./T_s
  Sum4 : Sum  Inputs=|+-
  x_a : Integrator  InitialConditionSource=external  InitialCondition=op_MGES.Subsystem_LPF1_x_a
  out : Outport
  wires:
  x_a/1 -> Sum4/2, out/1
  in/1 -> x_a/2, Sum4/1
  Sum4/1 -> Gain/1
  Gain/1 -> x_a/1

== system lib_AC_MGES/MGES/Subsystem/LPF2 ==
  in : Inport
  Gain : Gain  Gain=1./T_s
  Sum4 : Sum  Inputs=|+-
  x_a : Integrator  InitialConditionSource=external  InitialCondition=op_MGES.Subsystem_LPF2_x_a
  out : Outport
  wires:
  x_a/1 -> Sum4/2, out/1
  in/1 -> x_a/2, Sum4/1
  Sum4/1 -> Gain/1
  Gain/1 -> x_a/1

== system lib_AC_MGES/MGES/Subsystem/LPF3 ==
  in : Inport
  Gain : Gain  Gain=1./T_s
  Sum4 : Sum  Inputs=|+-
  x_a : Integrator  InitialConditionSource=external  InitialCondition=op_MGES.Subsystem_LPF3_x_a
  out : Outport
  wires:
  x_a/1 -> Sum4/2, out/1
  in/1 -> x_a/2, Sum4/1
  Sum4/1 -> Gain/1
  Gain/1 -> x_a/1

== system lib_AC_MGES/MGES/Subsystem/LPF4 ==
  in : Inport
  Gain : Gain  Gain=1./T_s
  Sum4 : Sum  Inputs=|+-
  x_a : Integrator  InitialConditionSource=external  InitialCondition=op_MGES.Subsystem_LPF4_x_a
  out : Outport
  wires:
  x_a/1 -> Sum4/2, out/1
  in/1 -> x_a/2, Sum4/1
  Sum4/1 -> Gain/1
  Gain/1 -> x_a/1

== system lib_AC_MGES/MGES/Subsystem/LPF7 ==
  in : Inport
  Gain : Gain  Gain=1./T_s
  Sum4 : Sum  Inputs=|+-
  x_a : Integrator  InitialConditionSource=external  InitialCondition=op_MGES.Subsystem_LPF7_x_a
  out : Outport
  wires:
  x_a/1 -> Sum4/2, out/1
  in/1 -> x_a/2, Sum4/1
  Sum4/1 -> Gain/1
  Gain/1 -> x_a/1

== system lib_AC_MGES/MGES/Subsystem1/Active ==
  In1 : Inport
  In2 : Inport  Port=2
  Impl : Subsystem  mask{K_P=K_P}
  Out1 : Outport
  wires:
  Impl/1(V_B) -> Out1/1
  In2/1 -> Impl/2(ifd)
  In1/1 -> Impl/1(vt)

== system lib_AC_MGES/MGES/Subsystem1/Bypass ==
  In1 : Inport
  In2 : Inport  Port=2
  Term1 : Terminator
  Term2 : Terminator
  Zero1 : Constant  Value=ones(1, length(block_buses))  VectorParams1D=off
  Out1 : Outport
  wires:
  Zero1/1 -> Out1/1
  In2/1 -> Term2/1
  In1/1 -> Term1/1

== system lib_AC_MGES/MGES/WOF_d2/Active ==
  In1 : Inport
  Impl : Subsystem
  Out1 : Outport
  wires:
  Impl/1(Out1) -> Out1/1
  In1/1 -> Impl/1(In1)

== system lib_AC_MGES/MGES/WOF_d2/Bypass ==
  In1 : Inport
  Out1 : Outport
  wires:
  In1/1 -> Out1/1

== system lib_AC_MGES/MGES/AVR_Vmeas_Filter1/Active/Impl ==
  in : Inport
  Gain : Gain  Gain=1./T_r
  Sum4 : Sum  Inputs=|+-
  x_a : Integrator  InitialConditionSource=external  InitialCondition=op_MGES.AVR_Vmeas_Filter1_Active_Impl_x_a
  out : Outport
  wires:
  Gain/1 -> x_a/1
  Sum4/1 -> Gain/1
  in/1 -> Sum4/1, x_a/2
  x_a/1 -> out/1, Sum4/2

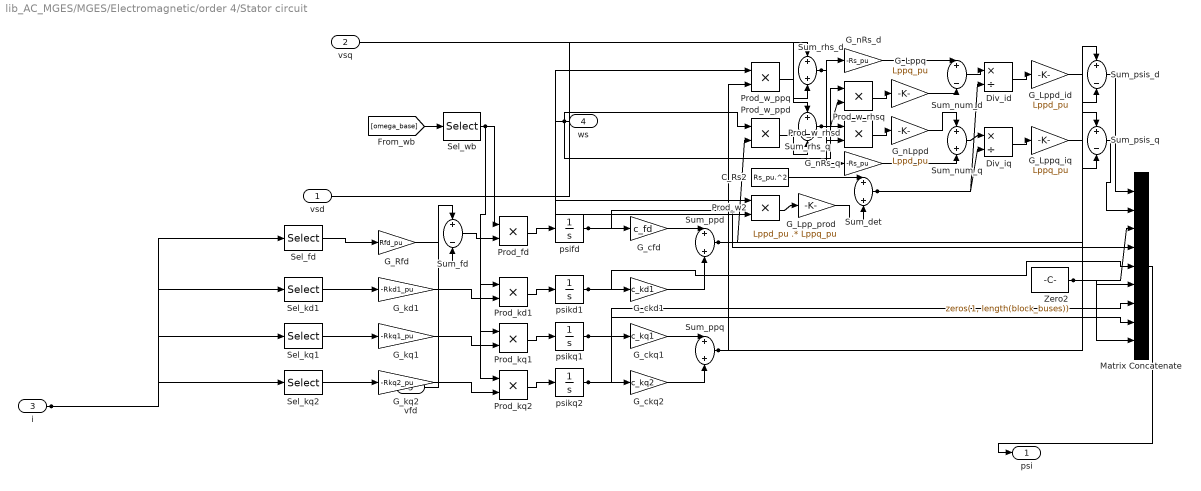
== system lib_AC_MGES/MGES/Electromagnetic/order 4/Stator circuit ==
  vsd : Inport
  vsq : Inport  Port=2
  i : Inport  Port=3
  ws : Inport  Port=4
  vfd : Inport  Port=5
  C_Rs2 : Constant  Value=Rs_pu.^2
  Div_id : Product  Inputs=*/
  Div_iq : Product  Inputs=*/
  G_Lpp_prod : Gain  Gain=Lppd_pu .* Lppq_pu
  G_Lppd_id : Gain  Gain=Lppd_pu
  G_Lppq : Gain  Gain=Lppq_pu
  G_Lppq_iq : Gain  Gain=Lppq_pu
  G_Rfd : Gain  Gain=Rfd_pu
  G_cfd : Gain  Gain=c_fd
  G_ckd1 : Gain  Gain=c_kd1
  G_ckq1 : Gain  Gain=c_kq1
  G_ckq2 : Gain  Gain=c_kq2
  G_kd1 : Gain  Gain=-Rkd1_pu
  G_kq1 : Gain  Gain=-Rkq1_pu
  G_kq2 : Gain  Gain=-Rkq2_pu
  G_nLppd : Gain  Gain=Lppd_pu
  G_nRs_d : Gain  Gain=-Rs_pu
  G_nRs_q : Gain  Gain=-Rs_pu
  Matrix Concatenate : Concatenate  NumInputs=9  Mode=Multidimensional array
  Prod_fd : Product  Inputs=**
  Prod_kd1 : Product  Inputs=**
  Prod_kq1 : Product  Inputs=**
  Prod_kq2 : Product  Inputs=**
  Prod_w2 : Product  Inputs=**
  Prod_w_ppd : Product  Inputs=**
  Prod_w_ppq : Product  Inputs=**
  Prod_w_rhsd : Product  Inputs=**
  Prod_w_rhsq : Product  Inputs=**
  Sel_fd : Selector  NumberOfDimensions=2  InputPortWidth=3  IndexOptions=Index vector (dialog),Select all  Indices=4,1  OutputSizes=1
  Sel_kd1 : Selector  NumberOfDimensions=2  InputPortWidth=3  IndexOptions=Index vector (dialog),Select all  Indices=5,1  OutputSizes=1
  Sel_kq1 : Selector  NumberOfDimensions=2  InputPortWidth=3  IndexOptions=Index vector (dialog),Select all  Indices=7,1  OutputSizes=1
  Sel_kq2 : Selector  NumberOfDimensions=2  InputPortWidth=3  IndexOptions=Index vector (dialog),Select all  Indices=8,1  OutputSizes=1
  Sel_wb : Selector  NumberOfDimensions=2  InputPortWidth=3  IndexOptions=Select all,Index vector (dialog)  Indices=1,block_fref  OutputSizes=1
  Sum_det : Sum
  Sum_fd : Sum  Inputs=+-
  Sum_num_d : Sum  Inputs=+-
  Sum_num_q : Sum
  Sum_ppd : Sum
  Sum_ppq : Sum
  Sum_psis_d : Sum  Inputs=+-
  Sum_psis_q : Sum  Inputs=+-
  Sum_rhs_d : Sum
  Sum_rhs_q : Sum  Inputs=+-
  Zero2 : Constant  Value=zeros(1, length(block_buses))  VectorParams1D=off
  psifd : Integrator  InitialCondition=op_MGES.Electromagnetic_order_4_Stator_circuit_psifd
  psikd1 : Integrator  InitialCondition=op_MGES.Electromagnetic_order_4_Stator_circuit_psikd1
  psikq1 : Integrator  InitialCondition=op_MGES.Electromagnetic_order_4_Stator_circuit_psikq1
  psikq2 : Integrator  InitialCondition=op_MGES.Electromagnetic_order_4_Stator_circuit_psikq2
  psi : Outport  VectorParamsAs1DForOutWhenUnconnected=off
  wires:
  [omega_base] -> Sel_wb/1
  vfd/1 -> Sum_fd/1
  G_Rfd/1 -> Sum_fd/2
  Sel_wb/1 -> Prod_fd/1, Prod_kd1/1, Prod_kq1/1, Prod_kq2/1
  Sum_fd/1 -> Prod_fd/2
  Prod_fd/1 -> psifd/1
  G_kd1/1 -> Prod_kd1/2
  Prod_kd1/1 -> psikd1/1
  G_kq1/1 -> Prod_kq1/2
  Prod_kq1/1 -> psikq1/1
  G_kq2/1 -> Prod_kq2/2
  Prod_kq2/1 -> psikq2/1
  psifd/1 -> G_cfd/1, Matrix Concatenate/4
  psikd1/1 -> G_ckd1/1, Matrix Concatenate/5
  G_cfd/1 -> Sum_ppd/1
  G_ckd1/1 -> Sum_ppd/2
  psikq1/1 -> G_ckq1/1, Matrix Concatenate/7
  psikq2/1 -> G_ckq2/1, Matrix Concatenate/8
  G_ckq1/1 -> Sum_ppq/1
  G_ckq2/1 -> Sum_ppq/2
  ws/1 -> Prod_w_ppq/1, Prod_w_ppd/1, Prod_w2/1, Prod_w2/2, Prod_w_rhsq/1, Prod_w_rhsd/1
  Sum_ppq/1 -> Prod_w_ppq/2, Sum_psis_q/1
  vsd/1 -> Sum_rhs_d/1
  Prod_w_ppq/1 -> Sum_rhs_d/2
  Sum_ppd/1 -> Prod_w_ppd/2, Sum_psis_d/1
  vsq/1 -> Sum_rhs_q/1
  Prod_w_ppd/1 -> Sum_rhs_q/2
  Prod_w2/1 -> G_Lpp_prod/1
  C_Rs2/1 -> Sum_det/1
  G_Lpp_prod/1 -> Sum_det/2
  Sum_rhs_d/1 -> G_nRs_d/1, Prod_w_rhsd/2
  Sum_rhs_q/1 -> Prod_w_rhsq/2, G_nRs_q/1
  Prod_w_rhsq/1 -> G_Lppq/1
  G_nRs_d/1 -> Sum_num_d/1
  G_Lppq/1 -> Sum_num_d/2
  Sum_num_d/1 -> Div_id/1
  Sum_det/1 -> Div_id/2, Div_iq/2
  Div_id/1 -> G_Lppd_id/1
  G_Lppd_id/1 -> Sum_psis_d/2
  Prod_w_rhsd/1 -> G_nLppd/1
  G_nLppd/1 -> Sum_num_q/1
  G_nRs_q/1 -> Sum_num_q/2
  Sum_num_q/1 -> Div_iq/1
  Div_iq/1 -> G_Lppq_iq/1
  G_Lppq_iq/1 -> Sum_psis_q/2
  Sum_psis_d/1 -> Matrix Concatenate/1
  Sum_psis_q/1 -> Matrix Concatenate/2
  Zero2/1 -> Matrix Concatenate/3, Matrix Concatenate/6, Matrix Concatenate/9
  Matrix Concatenate/1 -> psi/1
  i/1 -> Sel_fd/1, Sel_kd1/1, Sel_kq1/1, Sel_kq2/1
  Sel_fd/1 -> G_Rfd/1
  Sel_kd1/1 -> G_kd1/1
  Sel_kq1/1 -> G_kq1/1
  Sel_kq2/1 -> G_kq2/1

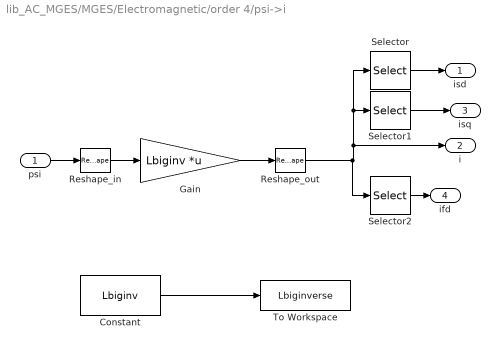
== system lib_AC_MGES/MGES/Electromagnetic/order 4/psi->i ==
  psi : Inport
  Constant : Constant  Value=Lbiginv
  Gain : Gain  Gain=Lbiginv  Multiplication=Matrix(K*u)
  Reshape_in : Reshape  OutputDimensionality=Column vector (2-D)
  Reshape_out : Reshape  OutputDimensionality=Customize  OutputDimensions=[9, length(block_buses)]
  Selector : Selector  NumberOfDimensions=2  InputPortWidth=9  IndexOptions=Index vector (dialog),Select all  Indices=[1],1  OutputSizes=1,1
  Selector1 : Selector  NumberOfDimensions=2  InputPortWidth=9  IndexOptions=Index vector (dialog),Select all  Indices=[2],1  OutputSizes=1,1
  Selector2 : Selector  NumberOfDimensions=2  InputPortWidth=9  IndexOptions=Index vector (dialog),Select all  Indices=4,1  OutputSizes=1,1
  To Workspace : ToWorkspace  VariableName=Lbiginverse  SaveFormat=Timeseries  SampleTime=-1
  isd : Outport  VectorParamsAs1DForOutWhenUnconnected=off
  i : Outport  Port=2  VectorParamsAs1DForOutWhenUnconnected=off
  isq : Outport  Port=3  VectorParamsAs1DForOutWhenUnconnected=off
  ifd : Outport  Port=4  VectorParamsAs1DForOutWhenUnconnected=off
  wires:
  Selector2/1 -> ifd/1
  Constant/1 -> To Workspace/1
  Selector1/1 -> isq/1
  Reshape_out/1 -> i/1, Selector/1, Selector1/1, Selector2/1
  Reshape_in/1 -> Gain/1
  psi/1 -> Reshape_in/1
  Gain/1 -> Reshape_out/1
  Selector/1 -> isd/1

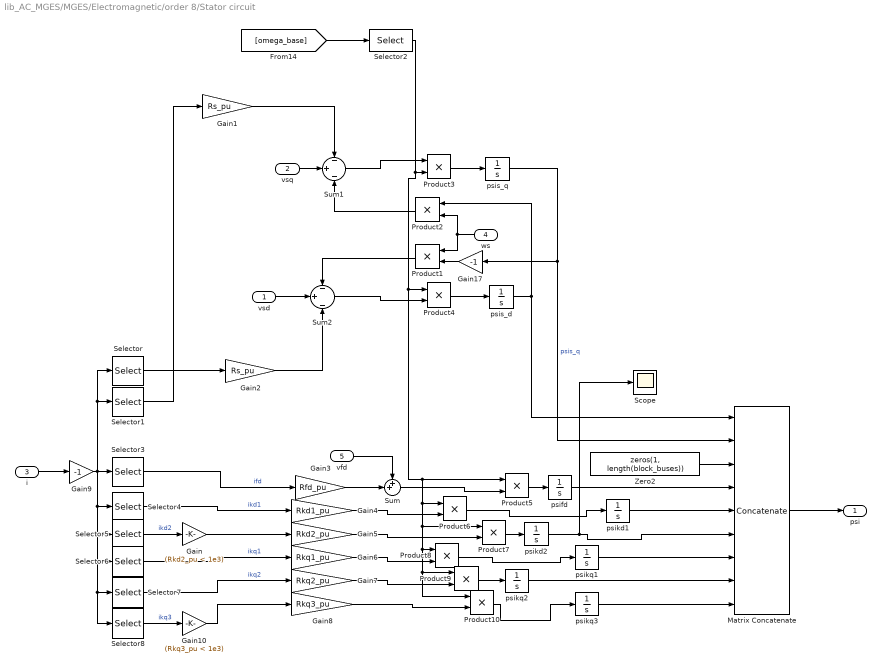
== system lib_AC_MGES/MGES/Electromagnetic/order 8/Stator circuit ==
  vsd : Inport
  vsq : Inport  Port=2
  i : Inport  Port=3
  ws : Inport  Port=4
  vfd : Inport  Port=5
  Gain : Gain  Gain=(Rkd2_pu < 1e3)
  Gain1 : Gain  Gain=Rs_pu
  Gain10 : Gain  Gain=(Rkq3_pu < 1e3)
  Gain17 : Gain  Gain=-1
  Gain2 : Gain  Gain=Rs_pu
  Gain3 : Gain  Gain=Rfd_pu
  Gain4 : Gain  Gain=Rkd1_pu
  Gain5 : Gain  Gain=Rkd2_pu
  Gain6 : Gain  Gain=Rkq1_pu
  Gain7 : Gain  Gain=Rkq2_pu
  Gain8 : Gain  Gain=Rkq3_pu
  Gain9 : Gain  Gain=-1
  Matrix Concatenate : Concatenate  NumInputs=9  Mode=Multidimensional array
  Product{1..10} (10 alike) : Product
  Scope : Scope
      settings: ActiveDisplayYMinimum=-1  ActiveDisplayYMaximum=1  DataLoggingVariableName=ScopeData14
  Selector : Selector  NumberOfDimensions=2  InputPortWidth=9  IndexOptions=Index vector (dialog),Select all  Indices=[1],1  OutputSizes=1,1
  Selector1 : Selector  NumberOfDimensions=2  InputPortWidth=9  IndexOptions=Index vector (dialog),Select all  Indices=[2],1  OutputSizes=1,1
  Selector2 : Selector  InputPortWidth=length(fref.ref_units)  IndexOptions=Index vector (dialog)  Indices=block_fref  OutputSizes=1
  Selector3 : Selector  NumberOfDimensions=2  InputPortWidth=9  IndexOptions=Index vector (dialog),Select all  Indices=[4],1  OutputSizes=1,1
  Selector4 : Selector  NumberOfDimensions=2  InputPortWidth=9  IndexOptions=Index vector (dialog),Select all  Indices=[5],1  OutputSizes=1,1
  Selector5 : Selector  NumberOfDimensions=2  InputPortWidth=9  IndexOptions=Index vector (dialog),Select all  Indices=[6],1  OutputSizes=1,1
  Selector6 : Selector  NumberOfDimensions=2  InputPortWidth=9  IndexOptions=Index vector (dialog),Select all  Indices=[7],1  OutputSizes=1,1
  Selector7 : Selector  NumberOfDimensions=2  InputPortWidth=9  IndexOptions=Index vector (dialog),Select all  Indices=[8],1  OutputSizes=1,1
  Selector8 : Selector  NumberOfDimensions=2  InputPortWidth=9  IndexOptions=Index vector (dialog),Select all  Indices=[9],1  OutputSizes=1,1
  Sum : Sum  Inputs=++|
  Sum1 : Sum  Inputs=-|+|-  InputSameDT=on  SaturateOnIntegerOverflow=on  OutDataTypeStr=Inherit: Same as first input
  Sum2 : Sum  Inputs=-|+|-  InputSameDT=on  SaturateOnIntegerOverflow=on  OutDataTypeStr=Inherit: Same as first input
  Zero2 : Constant  Value=zeros(1, length(block_buses))  VectorParams1D=off  OutDataTypeStr=Inherit: Inherit via back propagation
  psifd : Integrator  InitialCondition=op_MGES.Electromagnetic_order_8_Stator_circuit_psifd
  psikd1 : Integrator  InitialCondition=op_MGES.Electromagnetic_order_8_Stator_circuit_psikd1
  psikd2 : Integrator  InitialCondition=op_MGES.Electromagnetic_order_8_Stator_circuit_psikd2
  psikq1 : Integrator  InitialCondition=op_MGES.Electromagnetic_order_8_Stator_circuit_psikq1
  psikq2 : Integrator  InitialCondition=op_MGES.Electromagnetic_order_8_Stator_circuit_psikq2
  psikq3 : Integrator  InitialCondition=op_MGES.Electromagnetic_order_8_Stator_circuit_psikq3
  psis_d : Integrator  InitialCondition=op_MGES.Electromagnetic_order_8_Stator_circuit_psis_d
  psis_q : Integrator  InitialCondition=op_MGES.Electromagnetic_order_8_Stator_circuit_psis_q
  psi : Outport  VectorParamsAs1DForOutWhenUnconnected=off
  wires:
  Product3/1 -> psis_q/1
  Sum1/1 -> Product3/1
  Selector3/1 -> Gain3/1  "ifd"
  Selector8/1 -> Gain10/1  "ikq3"
  Selector7/1 -> Gain7/1  "ikq2"
  Selector6/1 -> Gain6/1  "ikq1"
  Selector5/1 -> Gain/1  "ikd2"
  Selector4/1 -> Gain4/1  "ikd1"
  Gain3/1 -> Sum/2
  vfd/1 -> Sum/1
  Sum/1 -> Product5/2
  Gain4/1 -> Product6/2
  Gain6/1 -> Product8/2
  Gain8/1 -> Product10/2
  Gain7/1 -> Product9/2
  psikq1/1 -> Matrix Concatenate/7
  psikd1/1 -> Matrix Concatenate/5
  Matrix Concatenate/1 -> psi/1
  i/1 -> Gain9/1
  Product6/1 -> psikd1/1
  Product7/1 -> psikd2/1
  Product8/1 -> psikq1/1
  Product9/1 -> psikq2/1
  Product10/1 -> psikq3/1
  Gain9/1 -> Selector8/1, Selector7/1, Selector6/1, Selector5/1, Selector4/1, Selector1/1, Selector/1, Selector3/1
  psikq2/1 -> Matrix Concatenate/8
  Zero2/1 -> Matrix Concatenate/3
  vsd/1 -> Sum2/2
  Sum2/1 -> Product4/2
  Product4/1 -> psis_d/1
  ws/1 -> Product1/1, Product2/2
  Gain17/1 -> Product1/2
  psis_q/1 -> Matrix Concatenate/2, Gain17/1  "psis_q"
  Product1/1 -> Sum2/1
  Product2/1 -> Sum1/3
  psis_d/1 -> Product2/1, Matrix Concatenate/1
  Selector/1 -> Gain2/1
  Gain2/1 -> Sum2/3
  Selector1/1 -> Gain1/1
  Gain1/1 -> Sum1/1
  vsq/1 -> Sum1/2
  [omega_base] -> Selector2/1
  Selector2/1 -> Product10/1, Product9/1, Product8/1, Product7/1, Product6/1, Product5/1, Product4/1, Product3/2
  Gain5/1 -> Product7/2
  psifd/1 -> Matrix Concatenate/4
  Product5/1 -> psifd/1
  psikd2/1 -> Matrix Concatenate/6, Scope/1
  psikq3/1 -> Matrix Concatenate/9
  Gain10/1 -> Gain8/1
  Gain/1 -> Gain5/1

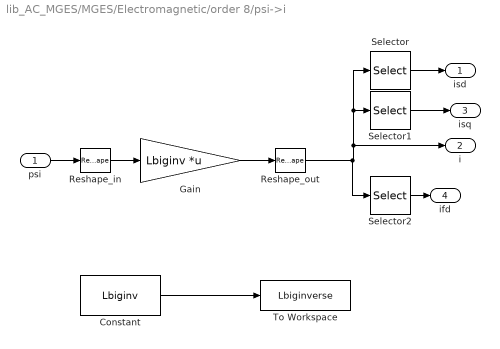
== system lib_AC_MGES/MGES/Electromagnetic/order 8/psi->i ==
  psi : Inport
  Constant : Constant  Value=Lbiginv
  Gain : Gain  Gain=Lbiginv  Multiplication=Matrix(K*u)
  Reshape_in : Reshape  OutputDimensionality=Column vector (2-D)
  Reshape_out : Reshape  OutputDimensionality=Customize  OutputDimensions=[9, length(block_buses)]
  Selector : Selector  NumberOfDimensions=2  InputPortWidth=9  IndexOptions=Index vector (dialog),Select all  Indices=[1],1  OutputSizes=1,1
  Selector1 : Selector  NumberOfDimensions=2  InputPortWidth=9  IndexOptions=Index vector (dialog),Select all  Indices=[2],1  OutputSizes=1,1
  Selector2 : Selector  NumberOfDimensions=2  InputPortWidth=9  IndexOptions=Index vector (dialog),Select all  Indices=4,1  OutputSizes=1,1
  To Workspace : ToWorkspace  VariableName=Lbiginverse  SaveFormat=Timeseries  SampleTime=-1
  isd : Outport  VectorParamsAs1DForOutWhenUnconnected=off
  i : Outport  Port=2  VectorParamsAs1DForOutWhenUnconnected=off
  isq : Outport  Port=3  VectorParamsAs1DForOutWhenUnconnected=off
  ifd : Outport  Port=4  VectorParamsAs1DForOutWhenUnconnected=off
  wires:
  Selector/1 -> isd/1
  Gain/1 -> Reshape_out/1
  psi/1 -> Reshape_in/1
  Reshape_in/1 -> Gain/1
  Reshape_out/1 -> Selector2/1, Selector1/1, Selector/1, i/1
  Selector1/1 -> isq/1
  Constant/1 -> To Workspace/1
  Selector2/1 -> ifd/1
